simulink model "Batt_Model"  (R2026a)
settings: Solver=FixedStepAuto  StopTime=1400  FixedStep=1
values from neighbouring files (symbols this model uses):
  Cd = 1350    [Batt_Cool.m]
  Cd_Pack = 810.5328    [Batt_Cool.m]
  Cell_Length = 0.227    [Batt_Cool.m]
  Cell_Volt = Cell_Data(:,2:3)    [Batt_Cool.m]
  Cell_Width = 0.226    [Batt_Cool.m]
  H_Convec = 5    [Batt_Cool.m]
  M_Pack = 150.2    [Batt_Cool.m]
  Np = 2    [Batt_Cool.m]
  Ns = 96    [Batt_Cool.m]
  R_Cell = [0.0117,0.0085,0.0090; 0.0110,0.0085,0.0090; 0.0114,0.0087,0.0092; 0.0107,0.0082,0.0088;0.0107,0.0083,0.0091; 0.0113,0.0085,0.0089; 0.0116,0.0085,0.0089]    [Batt_Cool.m]
  R_Inter = 0.0023    [Batt_Cool.m]
  SOC = [0;0.1;0.25;0.5;0.75;0.9;1.0]    [Batt_Cool.m]
  T_amb = 293.15    [Batt_Cool.m]
  T_amb_C = T_amb-273.15    (= 20)    [Batt_Cool.m]
  Temp = [278.15;293.15;313.15]    [Batt_Cool.m]
settings Model: Creator=sujee  LastModifiedBy=sujee

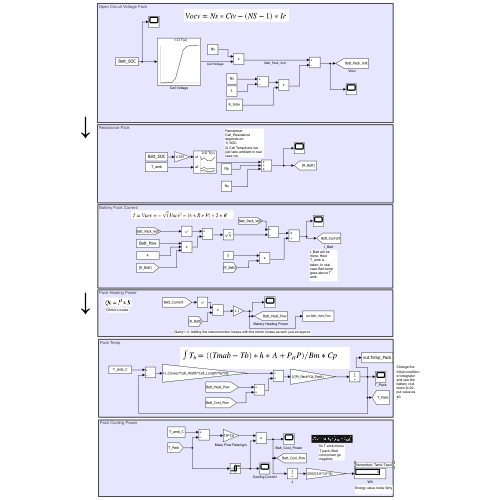
[thumbnail: Simulink's stored preview of the top-level diagram]
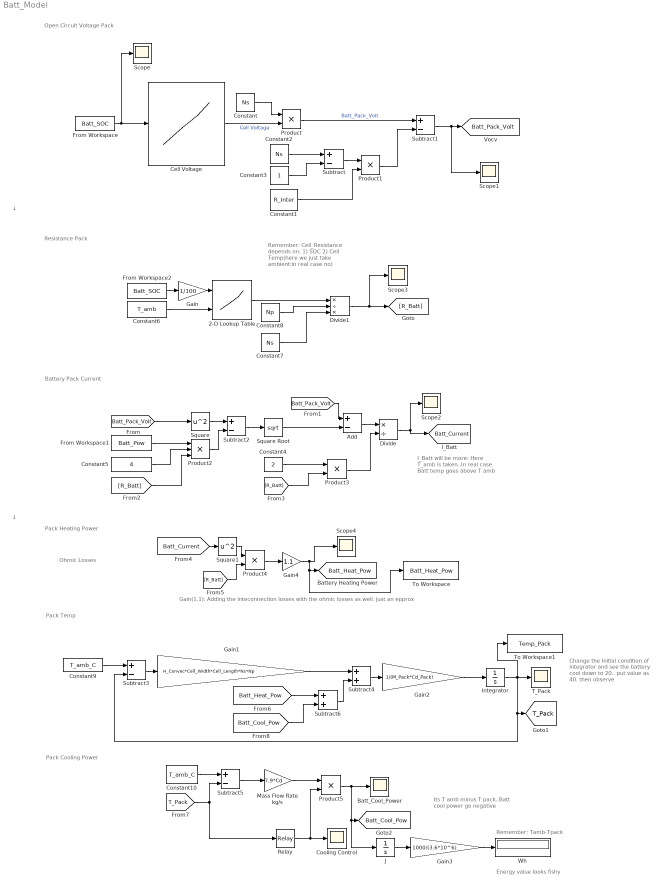
== system Batt_Model ==
  note: Remember: Tamb-Tpack
  note: Change the Initial condition of integrator and see the battery cool down to 20..
      | put value as 40.
      | then observe
  note: Energy value looks fishy
  note: Ohmic Losses
  note: Gain(1.1): Adding the inteconnection losses with the ohmic losses as well. just an epprox
  note: Pack Cooling Power
  note: Its T amb minus T pack..Batt cool power go negative
  note: Pack Temp
  note: ↓
  note: Pack Heating Power
  note: Battery Pack Current
  note: Resistance Pack
  note: I_Batt will be more: Here T_amb is taken..In real case Batt temp goes above T amb
  note: Remember:
      | Cell_Resistance depends on:
      | 1) SOC
      | 2) Cell Temp(here we just take ambient:in real case no)
  note: Open Circuit Voltage Pack
  note: ↓
  2-D Lookup Table : Lookup_n-D  BreakpointsForDimension1=SOC  BreakpointsForDimension2=Temp  Table=R_Cell  InternalRulePriority=Speed  RndMeth=Simplest
      settings: InputPortMap=u0,u1
  Add : Sum  Inputs=+-
  Batt_Cool_Power : Scope
      settings: ActiveDisplayYMinimum=-350752.8400113876  ActiveDisplayYMaximum=3.1567755601024888E+6  DataLoggingVariableName=ScopeData6
  Cell Voltage : Lookup_n-D  NumberOfTableDimensions=1  BreakpointsForDimension1=Cell_Volt(:,2)  Table=Cell_Volt(:,1)  InternalRulePriority=Speed  RndMeth=Simplest
  Constant : Constant  Value=Ns
  Constant1 : Constant  Value=R_Inter
  Constant10 : Constant  Value=T_amb_C
  Constant2 : Constant  Value=Ns
  Constant3 : Constant
  Constant4 : Constant  Value=2
  Constant5 : Constant  Value=4
  Constant6 : Constant  Value=T_amb
  Constant7 : Constant  Value=Ns
  Constant8 : Constant  Value=Np
  Constant9 : Constant  Value=T_amb_C
  Cooling Control : Scope
      settings: ActiveDisplayYMinimum=-1  ActiveDisplayYMaximum=1  DataLoggingVariableName=ScopeData7
  Divide : Product  Inputs=*/
  Divide1 : Product  Inputs=*/*
  From Workspace : FromWorkspace  VariableName=Batt_SOC
  From Workspace1 : FromWorkspace  VariableName=Batt_Pow
  From Workspace2 : FromWorkspace  VariableName=Batt_SOC
  Gain : Gain  Gain=1/100
  Gain1 : Gain  Gain=H_Convec*Cell_Width*Cell_Length*Ns*Np
  Gain2 : Gain  Gain=1/(M_Pack*Cd_Pack)
  Gain3 : Gain  Gain=1000/(3.6*10^6)
  Gain4 : Gain  Gain=1.1
  Integrator : Integrator  InitialCondition=T_amb_C
  J : Integrator
  Mass Flow Rate kg/s : Gain  Gain=7.9*Cd
  Product{,1,3..5} (5 alike) : Product
  Product2 : Product  Inputs=3
  Relay : Relay  OnSwitchValue=30  OffSwitchValue=20
  Scope{,1..4} (5 alike) : Scope
      Scope settings: ActiveDisplayYMinimum=96.9922045337588  ActiveDisplayYMaximum=98.977019641539641
      Scope1 settings: ActiveDisplayYMinimum=382.26950000000005  ActiveDisplayYMaximum=406.02949999999993
      Scope2 settings: ActiveDisplayYMinimum=-1  ActiveDisplayYMaximum=1  DataLoggingVariableName=ScopeData2
      Scope3 settings: ActiveDisplayYMinimum=0.30800000000000005  ActiveDisplayYMaximum=0.508  DataLoggingVariableName=ScopeData3
      Scope4 settings: ActiveDisplayYMinimum=-1  ActiveDisplayYMaximum=1  DataLoggingVariableName=ScopeData4
  Square : Math  Operator=square
  Square Root : Sqrt
  Square1 : Math  Operator=square
  Subtract{,1..3,5} (5 alike) : Sum  Inputs=+-
  Subtract4 : Sum
  Subtract6 : Sum
  T_Pack : Scope
      settings: ActiveDisplayYMinimum=19.9818431790254  ActiveDisplayYMaximum=20.163411388771408  DataLoggingVariableName=ScopeData5
  To Workspace : ToWorkspace  VariableName=Batt_Heat_Pow  SaveFormat=Timeseries  SampleTime=-1
  To Workspace1 : ToWorkspace  VariableName=Temp_Pack  SaveFormat=Timeseries  SampleTime=-1
  Wh : Display
  tag scope: Batt_Cool_Pow=global, Batt_Current=global, Batt_Heat_Pow=global, Batt_Pack_Volt=global, T_Pack=global
  wires:
  From Workspace/1 -> Cell Voltage/1, Scope/1
  Cell Voltage/1 -> Product/2  "Cell Voltage"
  Constant/1 -> Product/1
  Constant3/1 -> Subtract/2
  Constant2/1 -> Subtract/1
  Subtract/1 -> Product1/1
  Constant1/1 -> Product1/2
  Product/1 -> Subtract1/1  "Batt_Pack_Volt"
  Product1/1 -> Subtract1/2
  Subtract1/1 -> Scope1/1, [Batt_Pack_Volt]
  [Batt_Pack_Volt] -> Square/1
  Square/1 -> Subtract2/1
  Constant5/1 -> Product2/2
  From Workspace1/1 -> Product2/1
  Product2/1 -> Subtract2/2
  Subtract2/1 -> Square Root/1
  Constant6/1 -> 2-D Lookup Table/2
  From Workspace2/1 -> Gain/1
  Gain/1 -> 2-D Lookup Table/1
  2-D Lookup Table/1 -> Divide1/1
  Constant7/1 -> Divide1/3
  Constant8/1 -> Divide1/2
  Divide1/1 -> Scope3/1, [R_Batt]
  [R_Batt] -> Product2/3
  [Batt_Pack_Volt] -> Add/1
  Divide/1 -> [Batt_Current], Scope2/1
  Add/1 -> Divide/1
  [R_Batt] -> Product3/2
  Constant4/1 -> Product3/1
  Square Root/1 -> Add/2
  Product3/1 -> Divide/2
  [Batt_Current] -> Square1/1
  Square1/1 -> Product4/1
  [R_Batt] -> Product4/2
  Subtract3/1 -> Gain1/1
  Gain1/1 -> Subtract4/1
  Subtract4/1 -> Gain2/1
  Constant9/1 -> Subtract3/1
  Integrator/1 -> Subtract3/2, [T_Pack], To Workspace1/1, T_Pack/1
  Gain2/1 -> Integrator/1
  Constant10/1 -> Subtract5/1
  [T_Pack] -> Relay/1, Subtract5/2
  Subtract5/1 -> Mass Flow Rate kg/s/1
  Mass Flow Rate kg/s/1 -> Product5/1
  Relay/1 -> Cooling Control/1, Product5/2
  Product5/1 -> J/1, [Batt_Cool_Pow], Batt_Cool_Power/1
  [Batt_Heat_Pow] -> Subtract6/1
  [Batt_Cool_Pow] -> Subtract6/2
  Subtract6/1 -> Subtract4/2
  J/1 -> Gain3/1
  Gain3/1 -> Wh/1
  Product4/1 -> Gain4/1
  Gain4/1 -> Scope4/1, To Workspace/1, [Batt_Heat_Pow]
